simulink model "System_Model_Draft_2"  (R2025b)
settings: Solver=VariableStepAuto  StartTime=0.0  StopTime=10.0  RelTol=1e-3
model workspace (MAT data in the model file):
  I_Tensor = Simulink.Parameter
  I_Tensor.Complexity = 'real'
  I_Tensor.Dimensions = [3 3]
  I_Tensor.DataType = 'auto'
  I_xx = Simulink.Parameter
  I_xx.Complexity = 'real'
  I_xx.Dimensions = [0 0]
  I_xx.DataType = 'auto'
undefined symbols (not defined in the file or in its folder): Angle, Axis
libraries: robotcorelib x2
settings Model: Creator=User  LastModifiedBy=User

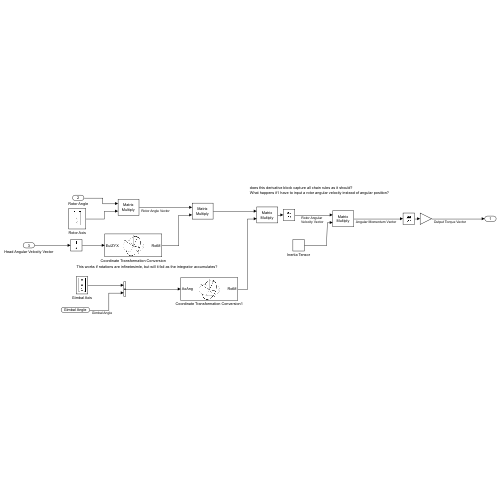
[thumbnail: Simulink's stored preview of the top-level diagram]
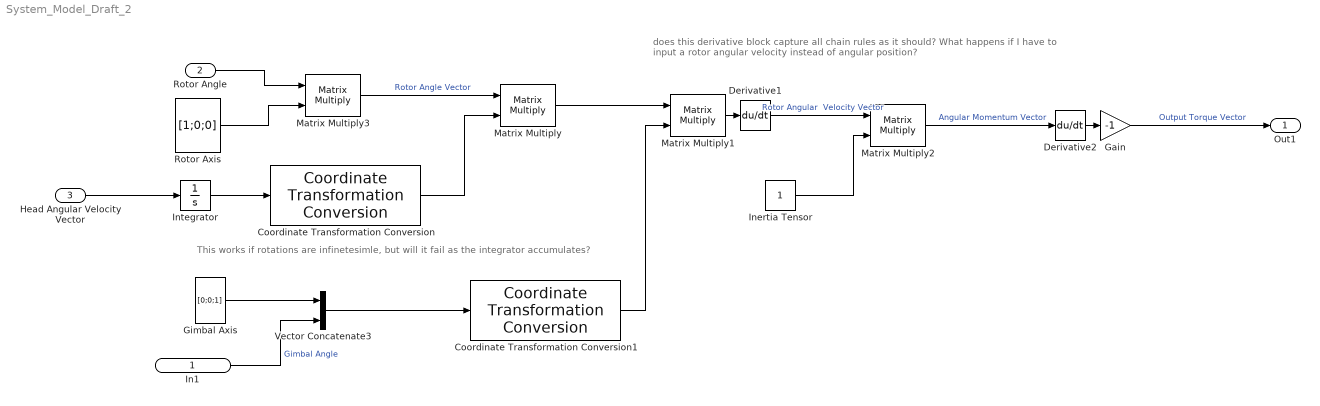
== system System_Model_Draft_2 ==
  note: does this derivative block capture all chain rules as it should?
      | What happens if I have to input a rotor angular velocity instead of angular position?
  note: This works if rotations are infinetesimle, but will it fail as the integrator accumulates?
  In1 : Inport
  Rotor Angle : Inport  Port=2
  Head Angular Velocity Vector : Inport  Port=3  PortDimensions=[1 3]
  Coordinate Transformation Conversion : robotcorelib/Coordinate Transformation Conversion  InputRepresentation=Euler Angles  InputEulerSequence=ZYX  ShowTrVecInputPort=on  OutputRepresentation=Rotation Matrix  OutputEulerSequence=ZYX  ShowTrVecOutputPort=on  SimulateUsing=Interpreted execution
  Coordinate Transformation Conversion1 : robotcorelib/Coordinate Transformation Conversion  InputRepresentation=Axis-Angle  InputEulerSequence=ZYX  ShowTrVecInputPort=on  OutputRepresentation=Rotation Matrix  OutputEulerSequence=ZYX  ShowTrVecOutputPort=on  SimulateUsing=Interpreted execution
  Derivative1 : Derivative
  Derivative2 : Derivative
  Gain : Gain  Gain=-1
  Gimbal Axis : Constant  Value=[0;0;1]  VectorParams1D=off
  Inertia Tensor : Constant
  Integrator : Integrator
  Matrix Multiply{,1..3} (4 alike) : Product  Multiplication=Matrix(*)
  Rotor Axis : Constant  Value=[1;0;0]  VectorParams1D=off
  Vector Concatenate3 : Concatenate
  Out1 : Outport
  wires:
  Vector Concatenate3/1 -> Coordinate Transformation Conversion1/1
  Gimbal Axis/1 -> Vector Concatenate3/1
  Rotor Axis/1 -> Matrix Multiply3/2
  Head Angular Velocity Vector/1 -> Integrator/1
  Rotor Angle/1 -> Matrix Multiply3/1
  Matrix Multiply3/1 -> Matrix Multiply/1  "Rotor Angle Vector"
  Integrator/1 -> Coordinate Transformation Conversion/1
  In1/1 -> Vector Concatenate3/2  "Gimbal Angle"
  Coordinate Transformation Conversion/1 -> Matrix Multiply/2
  Derivative1/1 -> Matrix Multiply2/1  "Rotor Angular  Velocity Vector"
  Matrix Multiply/1 -> Matrix Multiply1/1
  Coordinate Transformation Conversion1/1 -> Matrix Multiply1/2
  Matrix Multiply1/1 -> Derivative1/1
  Inertia Tensor/1 -> Matrix Multiply2/2
  Matrix Multiply2/1 -> Derivative2/1  "Angular Momentum Vector"
  Derivative2/1 -> Gain/1
  Gain/1 -> Out1/1  "Output Torque Vector"
